simulink model "ABS_Model"  (R2024b)
settings: Solver=ode45  StartTime=0.0  StopTime=5  RelTol=1e-3
undefined symbols (not defined in the file): J_R, m, M_B, r_R, v_0
libraries: simulink x1
settings Model: Creator=dinul  LastModifiedBy=Dinulkar

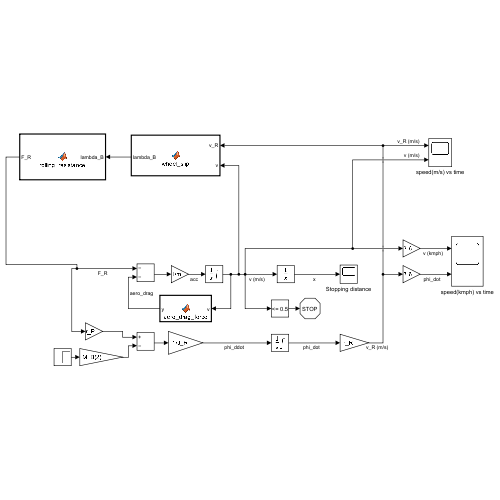
[thumbnail: Simulink's stored preview of the top-level diagram]
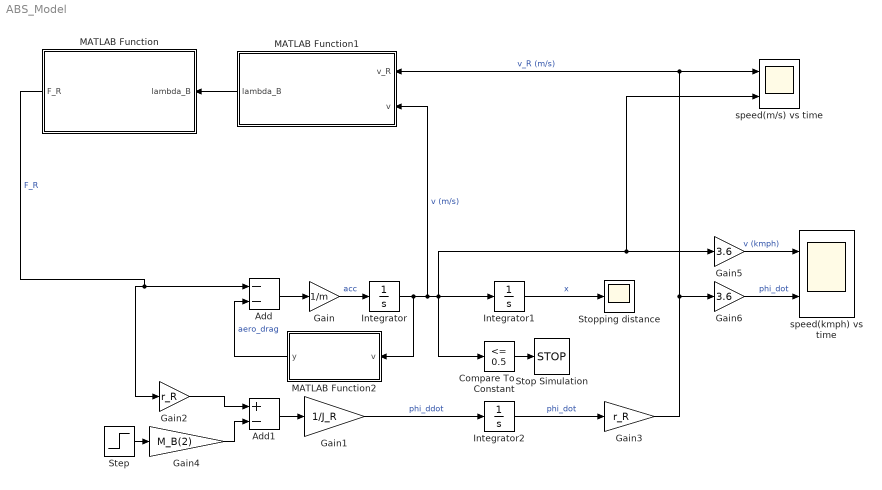
== system ABS_Model ==
  Add : Sum  Inputs=--
  Add1 : Sum  Inputs=+-
  Compare To Constant : simulink/Logic and Bit Operations/Compare To Constant  relop=<=  const=0.5  OutDataTypeStr=boolean
  Gain : Gain  Gain=1/m
  Gain1 : Gain  Gain=1/J_R
  Gain2 : Gain  Gain=r_R
  Gain3 : Gain  Gain=r_R
  Gain4 : Gain  Gain=M_B(2)
  Gain5 : Gain  Gain=3.6
  Gain6 : Gain  Gain=3.6
  Integrator : Integrator  InitialCondition=v_0  LimitOutput=on  LowerSaturationLimit=0
  Integrator1 : Integrator  LowerSaturationLimit=0
  Integrator2 : Integrator  InitialCondition=v_0/r_R  LimitOutput=on  LowerSaturationLimit=0
  MATLAB Function : MATLAB Function  TreatAsAtomicUnit=on
  MATLAB Function1 : MATLAB Function  TreatAsAtomicUnit=on
  MATLAB Function2 : MATLAB Function  TreatAsAtomicUnit=on
  Step : Step  SampleTime=0
  Stop Simulation : Stop
  Stopping distance : Scope
  speed(kmph) vs time : Scope  NumInputPorts=2
  speed(m/s) vs time : Scope  NumInputPorts=2
  wires:
  Gain/1 -> Integrator/1  "acc"
  Integrator/1 -> Compare To Constant/1, speed(m/s) vs time/2, Gain5/1, Integrator1/1, MATLAB Function1/2(v), MATLAB Function2/1(v)  "v (m/s)"
  MATLAB Function/1(F_R) -> Add/1, Gain2/1  "F_R"
  Add/1 -> Gain/1
  MATLAB Function2/1(y) -> Add/2  "aero_drag"
  Gain1/1 -> Integrator2/1  "phi_ddot"
  Add1/1 -> Gain1/1
  Gain2/1 -> Add1/1
  Integrator2/1 -> Gain3/1  "phi_dot"
  Integrator1/1 -> Stopping distance/1  "x"
  MATLAB Function1/1(lambda_B) -> MATLAB Function/1(lambda_B)
  Gain3/1 -> MATLAB Function1/1(v_R), speed(m/s) vs time/1, Gain6/1  "v_R (m/s)"
  Step/1 -> Gain4/1
  Gain4/1 -> Add1/2
  Compare To Constant/1 -> Stop Simulation/1
  Gain5/1 -> speed(kmph) vs time/1  "v (kmph)"
  Gain6/1 -> speed(kmph) vs time/2  "phi_dot"

== matlab function ABS_Model/MATLAB Function1 ==
  data: lambda_B output; v_R input; v input
function lambda_B = wheel_slip(v_R,v)

lambda_B = (v-v_R)/v;

== matlab function ABS_Model/MATLAB Function ==
  data: lambda_B input; F_R output
function F_R = rolling_resistance(lambda_B)
c1 = 0.86; c2 = 33.82; c3 = 0.36;
mu = (c1 * (1 - exp(-c2 * lambda_B)) - c3 * lambda_B);
g = 9.81;
m = 1500;
F_R = 1.5*mu*m*g;

== matlab function ABS_Model/MATLAB Function2 ==
  data: y output; v input
function y = aero_drag_force(v)
c_w = 0.3;
A = 2;
rho = 1.2;
y = c_w*A*rho*v^2/2;
